simulink model "gm_comm8qamtxrxhdl"  (R2025b)
settings: Solver=FixedStepDiscrete  StartTime=0.0  StopTime=20000*qam_params.symbolPeriod  RelTol=1e-3
PreLoadFcn:
  | qam_params = comm8qamtxrxhdl_init;
InitFcn:
  | qam_params = comm8qamtxrxhdl_init;
libraries: simulink x16, hdlmdlgenlib x7, hdlsllib x7, commchan3 x1, commrflib2 x1, dspsigops x1, dsphdlsigops2 x1, dspmlti4 x1, commdigbbndam3 x1, commsequence2 x1
(part 2 of 3)

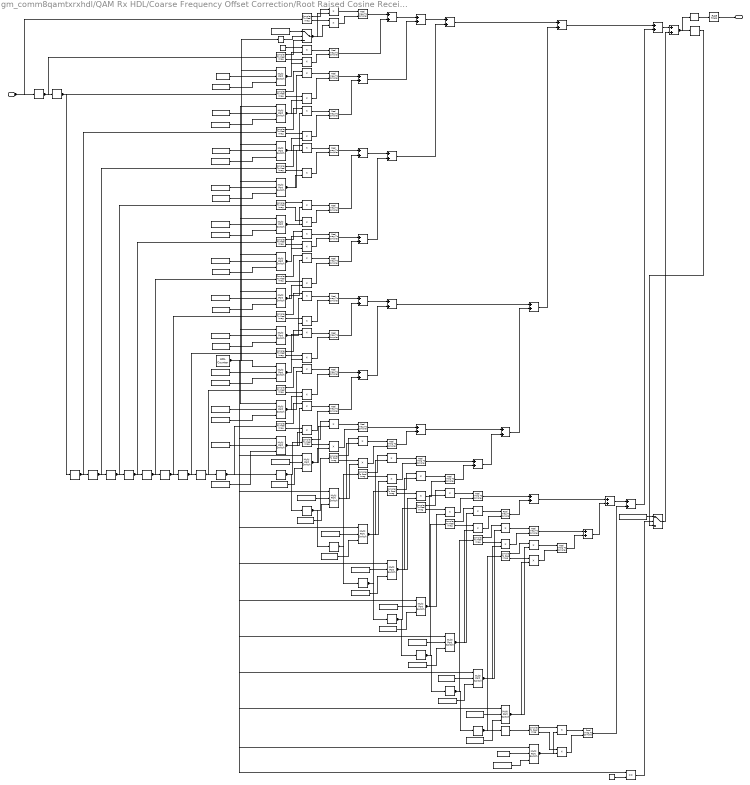
== system gm_comm8qamtxrxhdl/QAM Rx HDL/Coarse Frequency Offset Correction/Root Raised Cosine Receive Filter ==
  Root Raised Cosine Receive Filter_In : Inport  OutDataTypeStr=fixdt(1, 16, 15)  SampleTime=2.5e-07
      settings: SignalType=complex
  AddFeedback : Sum  OutDataTypeStr=fixdt(1, 16, 15)  SampleTime=2.5e-07
  Compare To Constant : simulink/Logic and Bit Operations/Compare To Constant  relop===  const=double(0)  OutDataTypeStr=boolean
  Constant : Constant  OutDataTypeStr=fixdt(0, 1, 0)  SampleTime=2.5e-07
  Constant1 : Constant  Value="fi(0,1,16,15,\"hex\",\"0000 + 0000 i\")"  OutDataTypeStr=fixdt(1, 16, 15)  SampleTime=2.5e-07
  Constant11 : Constant  Value=-0.0001678466796875  OutDataTypeStr=fixdt(1, 16, 16)  SampleTime=2.5e-07
  Constant12 : Constant  Value=0  OutDataTypeStr=fixdt(1, 16, 16)  SampleTime=2.5e-07
  Data Type Conversion : hdlmdlgenlib/Buffer
  Delay0 : Delay  DelayLength=double(1)  InitialCondition=0  SampleTime=2.5e-07
  Delay01 : Delay  DelayLength=double(2)  InitialCondition=0  SampleTime=2.5e-07
  Delay010 : Delay  DelayLength=double(2)  InitialCondition=0  SampleTime=2.5e-07
  Delay011 : Delay  DelayLength=double(2)  InitialCondition=0  SampleTime=2.5e-07
  Delay012 : Delay  DelayLength=double(2)  InitialCondition=0  SampleTime=2.5e-07
  Delay013 : Delay  DelayLength=double(2)  InitialCondition=0  SampleTime=2.5e-07
  Delay014 : Delay  DelayLength=double(2)  InitialCondition=0  SampleTime=2.5e-07
  Delay015 : Delay  DelayLength=double(2)  InitialCondition=0  SampleTime=2.5e-07
  Delay016 : Delay  DelayLength=double(2)  InitialCondition=0  SampleTime=2.5e-07
  Delay017 : Delay  DelayLength=double(2)  InitialCondition=0  SampleTime=2.5e-07
  Delay018 : Delay  DelayLength=double(2)  InitialCondition=0  SampleTime=2.5e-07
  Delay019 : Delay  DelayLength=double(2)  InitialCondition=0  SampleTime=2.5e-07
  Delay02 : Delay  DelayLength=double(2)  InitialCondition=0  SampleTime=2.5e-07
  Delay020 : Delay  DelayLength=double(1)  InitialCondition=0  SampleTime=2.5e-07
  Delay03 : Delay  DelayLength=double(2)  InitialCondition=0  SampleTime=2.5e-07
  Delay04 : Delay  DelayLength=double(2)  InitialCondition=0  SampleTime=2.5e-07
  Delay05 : Delay  DelayLength=double(2)  InitialCondition=0  SampleTime=2.5e-07
  Delay06 : Delay  DelayLength=double(2)  InitialCondition=0  SampleTime=2.5e-07
  Delay07 : Delay  DelayLength=double(2)  InitialCondition=0  SampleTime=2.5e-07
  Delay08 : Delay  DelayLength=double(2)  InitialCondition=0  SampleTime=2.5e-07
  Delay09 : Delay  DelayLength=double(2)  InitialCondition=0  SampleTime=2.5e-07
  HDL Counter : hdlsllib/Sources/HDL Counter  CountType=Count limited  CountInit=double(0)  CountStep=double(1)  CountMax=double(1)  CountFromType=Initial value  CountFrom=double(0)  CountResetPort=off  CountLoadPort=off  CountEnbPort=off  CountDirPort=off  CountHitOutputPort=off  CountDataType=Unsigned  CountWordLen=1  CountFracLen=0  CountSampTime=2.5e-07
  Multiport Switch{,1..19} (20 alike) : MultiPortSwitch  DataPortOrder=Zero-based contiguous  Inputs=2  DiagnosticForDefault=None  zeroidx=on  OutDataTypeStr=fixdt(1, 16, 16)  SampleTime=2.5e-07  SaturateOnIntegerOverflow=off  InputSameDT=off
  Product{10,101..109,1010..1041} (42 alike) : Product  Inputs=**  OutDataTypeStr=fixdt(1, 16, 15)  SampleTime=2.5e-07
  Product10_C2ReIm{,1..20} (21 alike) : ComplexToRealImag  SampleTime=2.5e-07
  Product10_ReIm2Complex{,1..20} (21 alike) : RealImagToComplex  SampleTime=2.5e-07
  Relational Operator : RelationalOperator  Operator===  OutDataTypeStr=fixdt(0, 1, 0)  SampleTime=2.5e-07  InputSameDT=off
  Switch : Switch  Criteria=u2 > Threshold  Threshold="fi(0,0,1,0,\"hex\",\"0\")"  OutDataTypeStr=fixdt(1, 16, 16)  SampleTime=2.5e-07  SaturateOnIntegerOverflow=off  InputSameDT=off
  Switch1 : Switch  Criteria=u2 > Threshold  Threshold="fi(0,0,1,0,\"hex\",\"0\")"  OutDataTypeStr=fixdt(1, 16, 15)  SampleTime=2.5e-07  SaturateOnIntegerOverflow=off  InputSameDT=off
  addtree{,1..19} (20 alike) : Sum  OutDataTypeStr=fixdt(1, 16, 15)  SampleTime=2.5e-07
  coeffSubVector : Constant  Value=-0.0041046142578125  OutDataTypeStr=fixdt(1, 16, 16)  SampleTime=2.5e-07
  coeffSubVector1 : Constant  Value=0.000762939453125  OutDataTypeStr=fixdt(1, 16, 16)  SampleTime=2.5e-07
  coeffSubVector10 : Constant  Value=-0.0391082763671875  OutDataTypeStr=fixdt(1, 16, 16)  SampleTime=2.5e-07
  coeffSubVector11 : Constant  Value=-0.026458740234375  OutDataTypeStr=fixdt(1, 16, 16)  SampleTime=2.5e-07
  coeffSubVector12 : Constant  Value=0.0391082763671875  OutDataTypeStr=fixdt(1, 16, 16)  SampleTime=2.5e-07
  coeffSubVector13 : Constant  Value=0.1443023681640625  OutDataTypeStr=fixdt(1, 16, 16)  SampleTime=2.5e-07
  coeffSubVector14 : Constant  Value=0.2430267333984375  OutDataTypeStr=fixdt(1, 16, 16)  SampleTime=2.5e-07
  coeffSubVector15 : Constant  Value=0.2834625244140625  OutDataTypeStr=fixdt(1, 16, 16)  SampleTime=2.5e-07
  coeffSubVector16 : Constant  Value=0.2430267333984375  OutDataTypeStr=fixdt(1, 16, 16)  SampleTime=2.5e-07
  coeffSubVector17 : Constant  Value=0.1443023681640625  OutDataTypeStr=fixdt(1, 16, 16)  SampleTime=2.5e-07
  coeffSubVector18 : Constant  Value=0.0391082763671875  OutDataTypeStr=fixdt(1, 16, 16)  SampleTime=2.5e-07
  coeffSubVector19 : Constant  Value=-0.026458740234375  OutDataTypeStr=fixdt(1, 16, 16)  SampleTime=2.5e-07
  coeffSubVector2 : Constant  Value=0.0041046142578125  OutDataTypeStr=fixdt(1, 16, 16)  SampleTime=2.5e-07
  coeffSubVector20 : Constant  Value=-0.0391082763671875  OutDataTypeStr=fixdt(1, 16, 16)  SampleTime=2.5e-07
  coeffSubVector21 : Constant  Value=-0.018707275390625  OutDataTypeStr=fixdt(1, 16, 16)  SampleTime=2.5e-07
  coeffSubVector{22,24,30,32} (4 alike) : Constant  Value=0.0038604736328125  OutDataTypeStr=fixdt(1, 16, 16)  SampleTime=2.5e-07
  coeffSubVector23 : Constant  Value=0.010589599609375  OutDataTypeStr=fixdt(1, 16, 16)  SampleTime=2.5e-07
  coeffSubVector25 : Constant  Value=-0.0037384033203125  OutDataTypeStr=fixdt(1, 16, 16)  SampleTime=2.5e-07
  coeffSubVector26 : Constant  Value=0.0041046142578125  OutDataTypeStr=fixdt(1, 16, 16)  SampleTime=2.5e-07
  coeffSubVector27 : Constant  Value=0.000762939453125  OutDataTypeStr=fixdt(1, 16, 16)  SampleTime=2.5e-07
  coeffSubVector28 : Constant  Value=-0.0041046142578125  OutDataTypeStr=fixdt(1, 16, 16)  SampleTime=2.5e-07
  coeffSubVector29 : Constant  Value=-0.0037384033203125  OutDataTypeStr=fixdt(1, 16, 16)  SampleTime=2.5e-07
  coeffSubVector3 : Constant  Value=0.0026702880859375  OutDataTypeStr=fixdt(1, 16, 16)  SampleTime=2.5e-07
  coeffSubVector31 : Constant  Value=0.010589599609375  OutDataTypeStr=fixdt(1, 16, 16)  SampleTime=2.5e-07
  coeffSubVector33 : Constant  Value=-0.018707275390625  OutDataTypeStr=fixdt(1, 16, 16)  SampleTime=2.5e-07
  coeffSubVector{4,6,34,36} (4 alike) : Constant  Value=-0.000946044921875  OutDataTypeStr=fixdt(1, 16, 16)  SampleTime=2.5e-07
  coeffSubVector35 : Constant  Value=-0.0025177001953125  OutDataTypeStr=fixdt(1, 16, 16)  SampleTime=2.5e-07
  coeffSubVector37 : Constant  Value=0.0026702880859375  OutDataTypeStr=fixdt(1, 16, 16)  SampleTime=2.5e-07
  coeffSubVector38 : Constant  Value=0.00146484375  OutDataTypeStr=fixdt(1, 16, 16)  SampleTime=2.5e-07
  coeffSubVector39 : Constant  Value=0.001251220703125  OutDataTypeStr=fixdt(1, 16, 16)  SampleTime=2.5e-07
  coeffSubVector5 : Constant  Value=-0.0025177001953125  OutDataTypeStr=fixdt(1, 16, 16)  SampleTime=2.5e-07
  coeffSubVector7 : Constant  Value=0.001251220703125  OutDataTypeStr=fixdt(1, 16, 16)  SampleTime=2.5e-07
  coeffSubVector8 : Constant  Value=0.00146484375  OutDataTypeStr=fixdt(1, 16, 16)  SampleTime=2.5e-07
  coeffSubVector9 : Constant  Value=-0.0001678466796875  OutDataTypeStr=fixdt(1, 16, 16)  SampleTime=2.5e-07
  rt : RateTransition  InitialCondition=double(0)  OutPortSampleTimeOpt=Multiple of input port sample time  OutPortSampleTimeMultiple=2
  Root Raised Cosine Receive Filter_out : Outport  OutDataTypeStr=fixdt(1, 16, 15)  SampleTime=5e-07
      settings: SignalType=complex
  wires:
  Switch1/1 -> AddFeedback/2
  Multiport Switch1/1 -> Product102/2, Product103/2
  Multiport Switch11/1 -> Product1022/2, Product1023/2
  Product1014/1 -> Product10_ReIm2Complex7/1
  Product1030/1 -> Product10_ReIm2Complex15/1
  coeffSubVector8/1 -> Multiport Switch4/2
  Product1040/1 -> Product10_ReIm2Complex20/1
  Constant1/1 -> Switch1/1
  Product1025/1 -> Product10_ReIm2Complex12/2
  Product1041/1 -> Product10_ReIm2Complex20/2
  Product1029/1 -> Product10_ReIm2Complex14/2
  Relational Operator/1 -> Switch1/2
  Product10_C2ReIm3/2 -> Product107/1
  Product10_C2ReIm19/1 -> Product1038/1
  Product10_C2ReIm3/1 -> Product106/1
  Product10_C2ReIm19/2 -> Product1039/1
  Product10_C2ReIm11/1 -> Product1022/1
  Product1037/1 -> Product10_ReIm2Complex18/2
  addtree3/1 -> addtree4/2
  Product105/1 -> Product10_ReIm2Complex2/2
  Product1021/1 -> Product10_ReIm2Complex10/2
  coeffSubVector5/1 -> Multiport Switch2/3
  Product10_ReIm2Complex12/1 -> addtree9/2
  Product10_C2ReIm18/1 -> Product1036/1
  Product10_C2ReIm2/2 -> Product105/1
  Product10_C2ReIm2/1 -> Product104/1
  Product10_C2ReIm18/2 -> Product1037/1
  Product10_C2ReIm12/1 -> Product1024/1
  Product10_C2ReIm4/1 -> Product108/1
  Product10_C2ReIm20/2 -> Product1041/1
  Product10_C2ReIm4/2 -> Product109/1
  Product10_C2ReIm20/1 -> Product1040/1
  Delay010/1 -> Delay011/1, Product10_C2ReIm8/1
  coeffSubVector39/1 -> Multiport Switch19/3
  Product1027/1 -> Product10_ReIm2Complex13/2
  Product1038/1 -> Product10_ReIm2Complex19/1
  Multiport Switch7/1 -> Product1015/2, Product1014/2
  coeffSubVector24/1 -> Multiport Switch12/2
  coeffSubVector16/1 -> Multiport Switch8/2
  Product1036/1 -> Product10_ReIm2Complex18/1
  Product1020/1 -> Product10_ReIm2Complex10/1
  coeffSubVector26/1 -> Multiport Switch13/2
  Multiport Switch/1 -> Product101/2, Product10/2
  Product10_ReIm2Complex17/1 -> addtree17/1
  coeffSubVector13/1 -> Multiport Switch6/3
  coeffSubVector21/1 -> Multiport Switch10/3
  Product1039/1 -> Product10_ReIm2Complex19/2
  Product10_ReIm2Complex7/1 -> addtree6/1
  HDL Counter/1 -> Multiport Switch/1, Relational Operator/1, Compare To Constant/1, Multiport Switch19/1, Multiport Switch17/1, Multiport Switch18/1, Multiport Switch14/1, Multiport Switch16/1, Multiport Switch5/1, Multiport Switch6/1, Multiport Switch8/1, Multiport Switch10/1, Multiport Switch13/1, Multiport Switch4/1, Multiport Switch2/1, Multiport Switch7/1, Multiport Switch3/1, Multiport Switch1/1, Multiport Switch12/1, Multiport Switch15/1, Multiport Switch11/1, Multiport Switch9/1
  Multiport Switch5/1 -> Product1011/2, Product1010/2
  addtree17/1 -> addtree18/2
  Product10_C2ReIm13/2 -> Product1027/1
  Product10_C2ReIm5/2 -> Product1011/1
  addtree4/1 -> AddFeedback/1
  Product1016/1 -> Product10_ReIm2Complex8/1
  Product1032/1 -> Product10_ReIm2Complex16/1
  Product103/1 -> Product10_ReIm2Complex1/2
  Product1035/1 -> Product10_ReIm2Complex17/2
  Product1019/1 -> Product10_ReIm2Complex9/2
  Product1028/1 -> Product10_ReIm2Complex14/1
  Product10_C2ReIm14/2 -> Product1029/1
  Delay012/1 -> Delay013/1, Product10_C2ReIm10/1
  Product1034/1 -> Product10_ReIm2Complex17/1
  Product10_C2ReIm15/1 -> Product1030/1
  addtree/1 -> addtree2/1
  Product10_C2ReIm15/2 -> Product1031/1
  Product10_C2ReIm7/2 -> Product1015/1
  coeffSubVector35/1 -> Multiport Switch17/3
  coeffSubVector28/1 -> Multiport Switch14/2
  Product10_C2ReIm9/1 -> Product1018/1
  Product10_C2ReIm1/2 -> Product103/1
  Product10_C2ReIm17/1 -> Product1034/1
  Product10_C2ReIm1/1 -> Product102/1
  Product10_C2ReIm17/2 -> Product1035/1
  Product1031/1 -> Product10_ReIm2Complex15/2
  Product1015/1 -> Product10_ReIm2Complex7/2
  coeffSubVector11/1 -> Multiport Switch5/3
  Product10_C2ReIm8/2 -> Product1017/1
  coeffSubVector19/1 -> Multiport Switch9/3
  Product10_C2ReIm/2 -> Product101/1
  Product10_C2ReIm16/1 -> Product1032/1
  Delay05/1 -> Product10_C2ReIm15/1, Delay06/1
  Product10_C2ReIm/1 -> Product10/1
  Product10_C2ReIm16/2 -> Product1033/1
  Product10_C2ReIm8/1 -> Product1016/1
  Product10_ReIm2Complex2/1 -> addtree1/1
  Root Raised Cosine Receive Filter_In/1 -> Delay0/1, Product10_C2ReIm20/1
  Product1033/1 -> Product10_ReIm2Complex16/2
  addtree18/1 -> addtree16/1
  Product1026/1 -> Product10_ReIm2Complex13/1
  addtree19/1 -> addtree18/1
  Product10_C2ReIm14/1 -> Product1028/1
  Product1017/1 -> Product10_ReIm2Complex8/2
  Product1023/1 -> Product10_ReIm2Complex11/2
  Product10_C2ReIm13/1 -> Product1026/1
  Multiport Switch17/1 -> Product1035/2, Product1034/2
  Product1024/1 -> Product10_ReIm2Complex12/1
  Product10_C2ReIm12/2 -> Product1025/1
  Product1022/1 -> Product10_ReIm2Complex11/1
  coeffSubVector29/1 -> Multiport Switch14/3
  Product10_C2ReIm11/2 -> Product1023/1
  coeffSubVector31/1 -> Multiport Switch15/3
  Product10_C2ReIm10/2 -> Product1021/1
  Product10_C2ReIm10/1 -> Product1020/1
  Delay09/1 -> Product10_C2ReIm7/1, Delay010/1
  Product1018/1 -> Product10_ReIm2Complex9/1
  Multiport Switch13/1 -> Product1027/2, Product1026/2
  Product10_C2ReIm9/2 -> Product1019/1
  Product10_C2ReIm7/1 -> Product1014/1
  Product1013/1 -> Product10_ReIm2Complex6/2
  Product1012/1 -> Product10_ReIm2Complex6/1
  addtree11/1 -> addtree12/2
  Product10_C2ReIm6/2 -> Product1013/1
  Product10_C2ReIm6/1 -> Product1012/1
  Product1011/1 -> Product10_ReIm2Complex5/2
  Product1010/1 -> Product10_ReIm2Complex5/1
  Product10_C2ReIm5/1 -> Product1010/1
  coeffSubVector27/1 -> Multiport Switch13/3
  Product109/1 -> Product10_ReIm2Complex4/2
  Product108/1 -> Product10_ReIm2Complex4/1
  Product107/1 -> Product10_ReIm2Complex3/2
  addtree7/1 -> addtree11/1
  Product106/1 -> Product10_ReIm2Complex3/1
  Product104/1 -> Product10_ReIm2Complex2/1
  addtree10/1 -> addtree11/2
  Product102/1 -> Product10_ReIm2Complex1/1
  coeffSubVector30/1 -> Multiport Switch15/2
  Product101/1 -> Product10_ReIm2Complex/2
  Product10/1 -> Product10_ReIm2Complex/1
  Product10_ReIm2Complex18/1 -> addtree17/2
  addtree16/1 -> addtree12/1
  coeffSubVector2/1 -> Multiport Switch1/2
  Product10_ReIm2Complex8/1 -> addtree6/2
  addtree14/1 -> addtree15/2
  Product10_ReIm2Complex16/1 -> addtree14/2
  Delay017/1 -> Delay018/1, Product10_C2ReIm2/1
  Product10_ReIm2Complex15/1 -> addtree14/1
  Product10_ReIm2Complex3/1 -> addtree1/2
  Multiport Switch3/1 -> Product106/2, Product107/2
  Product10_ReIm2Complex9/1 -> addtree8/1
  addtree13/1 -> addtree15/1
  Delay01/1 -> Product10_C2ReIm17/1, Delay02/1
  Product10_ReIm2Complex14/1 -> addtree13/2
  Product10_ReIm2Complex13/1 -> addtree13/1
  addtree6/1 -> addtree7/2
  addtree9/1 -> addtree10/2
  Product10_ReIm2Complex10/1 -> addtree8/2
  addtree5/1 -> addtree7/1
  Product10_ReIm2Complex6/1 -> addtree5/2
  Product10_ReIm2Complex5/1 -> addtree5/1
  addtree2/1 -> addtree3/1
  addtree1/1 -> addtree2/2
  Product10_ReIm2Complex1/1 -> addtree/2
  rt/1 -> Root Raised Cosine Receive Filter_out/1
  Compare To Constant/1 -> Switch/2
  Constant12/1 -> Switch/3
  Constant11/1 -> Switch/1
  Multiport Switch8/1 -> Product1017/2, Product1016/2
  Multiport Switch12/1 -> Product1025/2, Product1024/2
  Product10_ReIm2Complex20/1 -> addtree19/1
  coeffSubVector25/1 -> Multiport Switch12/3
  coeffSubVector38/1 -> Multiport Switch19/2
  coeffSubVector37/1 -> Multiport Switch18/3
  coeffSubVector36/1 -> Multiport Switch18/2
  Product10_ReIm2Complex11/1 -> addtree9/1
  coeffSubVector34/1 -> Multiport Switch17/2
  coeffSubVector3/1 -> Multiport Switch1/3
  coeffSubVector33/1 -> Multiport Switch16/3
  coeffSubVector32/1 -> Multiport Switch16/2
  coeffSubVector14/1 -> Multiport Switch7/2
  coeffSubVector23/1 -> Multiport Switch11/3
  Multiport Switch9/1 -> Product1019/2, Product1018/2
  coeffSubVector22/1 -> Multiport Switch11/2
  coeffSubVector12/1 -> Multiport Switch6/2
  coeffSubVector20/1 -> Multiport Switch10/2
  coeffSubVector18/1 -> Multiport Switch9/2
  Delay03/1 -> Delay04/1, Product10_C2ReIm13/1
  coeffSubVector17/1 -> Multiport Switch8/3
  coeffSubVector15/1 -> Multiport Switch7/3
  Multiport Switch10/1 -> Product1021/2, Product1020/2
  Data Type Conversion/1 -> rt/1
  coeffSubVector10/1 -> Multiport Switch5/2
  coeffSubVector9/1 -> Multiport Switch4/3
  coeffSubVector7/1 -> Multiport Switch3/3
  coeffSubVector6/1 -> Multiport Switch3/2
  Multiport Switch6/1 -> Product1012/2, Product1013/2
  AddFeedback/1 -> Data Type Conversion/1, Delay020/1
  coeffSubVector4/1 -> Multiport Switch2/2
  coeffSubVector1/1 -> Multiport Switch/3
  coeffSubVector/1 -> Multiport Switch/2
  Constant/1 -> Relational Operator/2
  Delay019/1 -> Product10_C2ReIm4/1
  Switch/1 -> Product1041/2, Product1040/2
  Multiport Switch19/1 -> Product1039/2, Product1038/2
  Multiport Switch18/1 -> Product1037/2, Product1036/2
  Multiport Switch16/1 -> Product1033/2, Product1032/2
  Multiport Switch15/1 -> Product1031/2, Product1030/2
  Multiport Switch14/1 -> Product1029/2, Product1028/2
  Delay011/1 -> Delay012/1, Product10_C2ReIm9/1
  Delay013/1 -> Delay014/1, Product10_C2ReIm11/1
  Multiport Switch4/1 -> Product109/2, Product108/2
  Delay015/1 -> Delay016/1, Product10_C2ReIm/1
  Multiport Switch2/1 -> Product105/2, Product104/2
  Delay018/1 -> Product10_C2ReIm3/1, Delay019/1
  Delay016/1 -> Product10_C2ReIm1/1, Delay017/1
  Delay014/1 -> Product10_C2ReIm12/1, Delay015/1
  Delay06/1 -> Product10_C2ReIm16/1, Delay07/1
  Delay08/1 -> Product10_C2ReIm6/1, Delay09/1
  Delay07/1 -> Product10_C2ReIm5/1, Delay08/1
  Delay04/1 -> Product10_C2ReIm14/1, Delay05/1
  Delay02/1 -> Product10_C2ReIm18/1, Delay03/1
  Delay0/1 -> Product10_C2ReIm19/1, Delay01/1
  addtree15/1 -> addtree16/2
  addtree12/1 -> addtree4/1
  Product10_ReIm2Complex19/1 -> addtree19/2
  addtree8/1 -> addtree10/1
  Product10_ReIm2Complex/1 -> addtree/1
  Product10_ReIm2Complex4/1 -> addtree3/2
  Delay020/1 -> Switch1/3

== system gm_comm8qamtxrxhdl/QAM Rx HDL/Demodulate/Rectangular QAM Demodulator Baseband ==
  u : Inport  OutDataTypeStr=fixdt(1, 16, 12)  PortDimensions=1  SampleTime=5e-07
      settings: SignalType=complex
  Rectangular QAM Demodulator Baseband : MATLAB Function  TreatAsAtomicUnit=on
  y : Outport  SampleTime=5e-07
  wires:
  u/1 -> Rectangular QAM Demodulator Baseband/1(u)
  Rectangular QAM Demodulator Baseband/1(y) -> y/1

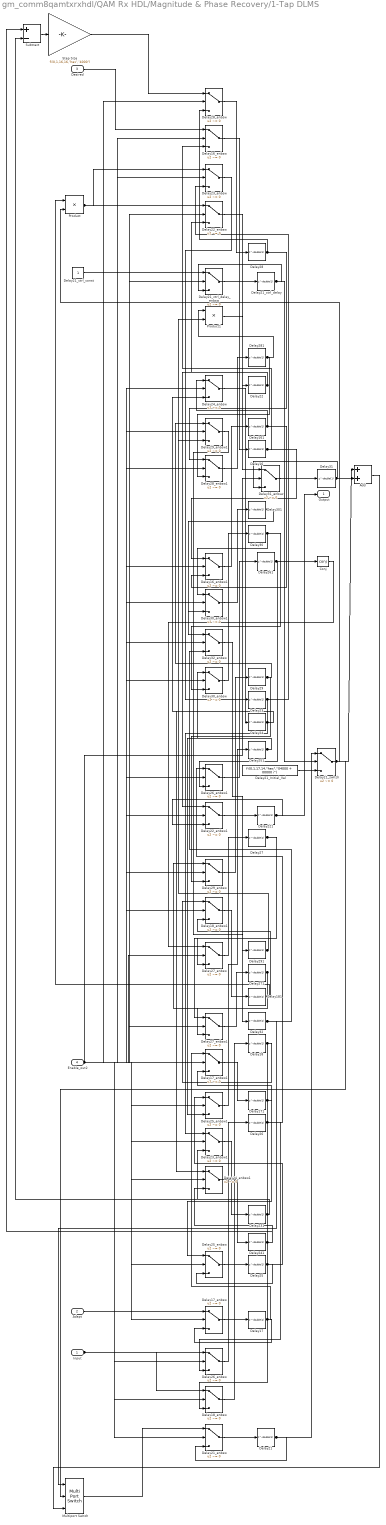
== system gm_comm8qamtxrxhdl/QAM Rx HDL/Magnitude & Phase Recovery/1-Tap DLMS ==
  Input : Inport  OutDataTypeStr=fixdt(1, 16, 15)  PortDimensions=1  SampleTime=5e-07
      settings: SignalType=complex
  Adapt : Inport  Port=2  OutDataTypeStr=boolean  PortDimensions=1  SampleTime=5e-07
  Desired : Inport  Port=3  OutDataTypeStr=fixdt(1, 16, 15)  PortDimensions=1  SampleTime=5e-07
      settings: SignalType=complex
  Enable_out2 : Inport  Port=4  OutDataTypeStr=boolean  SampleTime=5e-07
  Add : Sum  OutDataTypeStr=fixdt(1, 17, 14)  AccumDataTypeStr=fixdt(1, 19, 15)  SampleTime=5e-07
  Conj : Math  Operator=conj  SignedPower=on  OutDataTypeStr=fixdt(1, 16, 15)
  Delay{16..18,21..32,161,171,181,221,231,241,251,261,271,281,291,301} (27 alike) : Delay  DelayLength=double(1)  InitialCondition=0
  Delay16_enbsw : Switch  Criteria=u2 ~= 0  Threshold=double(0)  OutDataTypeStr=fixdt(1, 16, 15)  SampleTime=5e-07  SaturateOnIntegerOverflow=off  InputSameDT=off
  Delay16_enbsw1 : Switch  Criteria=u2 ~= 0  Threshold=double(0)  OutDataTypeStr=fixdt(1, 16, 15)  SampleTime=5e-07  SaturateOnIntegerOverflow=off  InputSameDT=off
  Delay17_enbsw : Switch  Criteria=u2 ~= 0  Threshold=double(0)  OutDataTypeStr=boolean  SampleTime=5e-07  SaturateOnIntegerOverflow=off  InputSameDT=off
  Delay17_enbsw1 : Switch  Criteria=u2 ~= 0  Threshold=double(0)  OutDataTypeStr=boolean  SampleTime=5e-07  SaturateOnIntegerOverflow=off  InputSameDT=off
  Delay18_enbsw : Switch  Criteria=u2 ~= 0  Threshold=double(0)  OutDataTypeStr=fixdt(1, 16, 15)  SampleTime=5e-07  SaturateOnIntegerOverflow=off  InputSameDT=off
  Delay18_enbsw1 : Switch  Criteria=u2 ~= 0  Threshold=double(0)  OutDataTypeStr=fixdt(1, 16, 15)  SampleTime=5e-07  SaturateOnIntegerOverflow=off  InputSameDT=off
  Delay21_Initial_Val : Constant  Value="fi(0,1,17,14,\"hex\",\"04000 + 00000 i\")"  OutDataTypeStr=fixdt(1, 17, 14)  SampleTime=5e-07
  Delay21_ctrl_const : Constant  OutDataTypeStr=boolean  SampleTime=5e-07
  Delay21_ctrl_delay : Delay  DelayLength=double(1)  InitialCondition=0
  Delay21_ctrl_delay_enbsw : Switch  Criteria=u2 ~= 0  Threshold=double(0)  OutDataTypeStr=boolean  SampleTime=5e-07  SaturateOnIntegerOverflow=off  InputSameDT=off
  Delay21_enbsw : Switch  Criteria=u2 ~= 0  Threshold=double(0)  OutDataTypeStr=fixdt(1, 17, 14)  SampleTime=5e-07  SaturateOnIntegerOverflow=off  InputSameDT=off
  Delay21_switch : Switch  Criteria=u2 ~= 0  Threshold=double(0)  OutDataTypeStr=fixdt(1, 17, 14)  SampleTime=5e-07  SaturateOnIntegerOverflow=off  InputSameDT=off
  Delay22_enbsw : Switch  Criteria=u2 ~= 0  Threshold=double(0)  OutDataTypeStr=fixdt(1, 16, 14)  SampleTime=5e-07  SaturateOnIntegerOverflow=off  InputSameDT=off
  Delay22_enbsw1 : Switch  Criteria=u2 ~= 0  Threshold=double(0)  OutDataTypeStr=fixdt(1, 16, 14)  SampleTime=5e-07  SaturateOnIntegerOverflow=off  InputSameDT=off
  Delay23_enbsw : Switch  Criteria=u2 ~= 0  Threshold=double(0)  OutDataTypeStr=fixdt(1, 16, 14)  SampleTime=5e-07  SaturateOnIntegerOverflow=off  InputSameDT=off
  Delay23_enbsw1 : Switch  Criteria=u2 ~= 0  Threshold=double(0)  OutDataTypeStr=fixdt(1, 16, 14)  SampleTime=5e-07  SaturateOnIntegerOverflow=off  InputSameDT=off
  Delay24_enbsw : Switch  Criteria=u2 ~= 0  Threshold=double(0)  OutDataTypeStr=fixdt(1, 16, 15)  SampleTime=5e-07  SaturateOnIntegerOverflow=off  InputSameDT=off
  Delay24_enbsw1 : Switch  Criteria=u2 ~= 0  Threshold=double(0)  OutDataTypeStr=fixdt(1, 16, 15)  SampleTime=5e-07  SaturateOnIntegerOverflow=off  InputSameDT=off
  Delay25_enbsw : Switch  Criteria=u2 ~= 0  Threshold=double(0)  OutDataTypeStr=boolean  SampleTime=5e-07  SaturateOnIntegerOverflow=off  InputSameDT=off
  Delay25_enbsw1 : Switch  Criteria=u2 ~= 0  Threshold=double(0)  OutDataTypeStr=boolean  SampleTime=5e-07  SaturateOnIntegerOverflow=off  InputSameDT=off
  Delay26_enbsw : Switch  Criteria=u2 ~= 0  Threshold=double(0)  OutDataTypeStr=fixdt(1, 16, 15)  SampleTime=5e-07  SaturateOnIntegerOverflow=off  InputSameDT=off
  Delay26_enbsw1 : Switch  Criteria=u2 ~= 0  Threshold=double(0)  OutDataTypeStr=fixdt(1, 16, 15)  SampleTime=5e-07  SaturateOnIntegerOverflow=off  InputSameDT=off
  Delay27_enbsw : Switch  Criteria=u2 ~= 0  Threshold=double(0)  OutDataTypeStr=fixdt(1, 16, 15)  SampleTime=5e-07  SaturateOnIntegerOverflow=off  InputSameDT=off
  Delay27_enbsw1 : Switch  Criteria=u2 ~= 0  Threshold=double(0)  OutDataTypeStr=fixdt(1, 16, 15)  SampleTime=5e-07  SaturateOnIntegerOverflow=off  InputSameDT=off
  Delay28_enbsw : Switch  Criteria=u2 ~= 0  Threshold=double(0)  OutDataTypeStr=fixdt(1, 16, 15)  SampleTime=5e-07  SaturateOnIntegerOverflow=off  InputSameDT=off
  Delay28_enbsw1 : Switch  Criteria=u2 ~= 0  Threshold=double(0)  OutDataTypeStr=fixdt(1, 16, 15)  SampleTime=5e-07  SaturateOnIntegerOverflow=off  InputSameDT=off
  Delay29_enbsw : Switch  Criteria=u2 ~= 0  Threshold=double(0)  OutDataTypeStr=fixdt(1, 16, 15)  SampleTime=5e-07  SaturateOnIntegerOverflow=off  InputSameDT=off
  Delay29_enbsw1 : Switch  Criteria=u2 ~= 0  Threshold=double(0)  OutDataTypeStr=fixdt(1, 16, 15)  SampleTime=5e-07  SaturateOnIntegerOverflow=off  InputSameDT=off
  Delay30_enbsw : Switch  Criteria=u2 ~= 0  Threshold=double(0)  OutDataTypeStr=boolean  SampleTime=5e-07  SaturateOnIntegerOverflow=off  InputSameDT=off
  Delay30_enbsw1 : Switch  Criteria=u2 ~= 0  Threshold=double(0)  OutDataTypeStr=boolean  SampleTime=5e-07  SaturateOnIntegerOverflow=off  InputSameDT=off
  Delay31_enbsw : Switch  Criteria=u2 ~= 0  Threshold=double(0)  OutDataTypeStr=fixdt(1, 16, 15)  SampleTime=5e-07  SaturateOnIntegerOverflow=off  InputSameDT=off
  Delay32_enbsw : Switch  Criteria=u2 ~= 0  Threshold=double(0)  OutDataTypeStr=boolean  SampleTime=5e-07  SaturateOnIntegerOverflow=off  InputSameDT=off
  Multiport Switch : MultiPortSwitch  DataPortOrder=Zero-based contiguous  Inputs=2  DiagnosticForDefault=None  zeroidx=on  OutDataTypeStr=fixdt(1, 17, 14)  SampleTime=5e-07  SaturateOnIntegerOverflow=off  InputSameDT=off
  Product : Product  Inputs=**  OutDataTypeStr=fixdt(1, 16, 14)  SampleTime=5e-07
  Product1 : Product  Inputs=**  OutDataTypeStr=fixdt(1, 16, 15)  SampleTime=5e-07
  Step Size : Gain  Gain="fi(0,1,16,16,\"hex\",\"4000\")"  ParamDataTypeStr=fixdt(1, 16, 16)  OutDataTypeStr=fixdt(1, 16, 15)  SampleTime=5e-07
  Subtract : Sum  Inputs=+-  OutDataTypeStr=fixdt(1, 16, 14)  AccumDataTypeStr=fixdt(1, 16, 14)  SampleTime=5e-07
  Output : Outport  SampleTime=5e-07  VectorParamsAs1DForOutWhenUnconnected=off
  wires:
  Input/1 -> Delay18_enbsw/1, Delay26_enbsw/1
  Subtract/1 -> Step Size/1
  Delay22_enbsw/1 -> Delay22/1
  Desired/1 -> Delay16_enbsw/1
  Adapt/1 -> Delay17_enbsw/1
  Step Size/1 -> Delay28_enbsw/1
  Product/1 -> Delay23_enbsw/1, Delay22_enbsw/1
  Delay221/1 -> Delay22_enbsw1/3, Output/1
  Delay21_Initial_Val/1 -> Delay21_switch/3
  Delay21_ctrl_const/1 -> Delay21_ctrl_delay_enbsw/1
  Delay22/1 -> Delay22_enbsw/3, Delay22_enbsw1/1
  Enable_out2/1 -> Delay31_enbsw/2, Delay22_enbsw1/2, Delay32_enbsw/2, Delay26_enbsw/2, Delay26_enbsw1/2, Delay29_enbsw/2, Delay27_enbsw1/2, Delay24_enbsw1/2, Delay27_enbsw/2, Delay16_enbsw/2, Delay23_enbsw/2, Delay21_enbsw/2, Delay30_enbsw/2, Delay16_enbsw1/2, Delay22_enbsw/2, Delay17_enbsw1/2, Delay25_enbsw/2, Delay17_enbsw/2, Delay23_enbsw1/2, Delay18_enbsw/2, Delay21_ctrl_delay_enbsw/2, Delay28_enbsw/2, Delay30_enbsw1/2, Delay29_enbsw1/2, Delay18_enbsw1/2, Delay28_enbsw1/2, Delay24_enbsw/2, Delay25_enbsw1/2
  Multiport Switch/1 -> Delay21_enbsw/1
  Delay28_enbsw/1 -> Delay28/1
  Delay16_enbsw/1 -> Delay16/1
  Delay23_enbsw/1 -> Delay23/1
  Delay21_ctrl_delay_enbsw/1 -> Delay21_ctrl_delay/1
  Product1/1 -> Delay31_enbsw/1
  Delay24_enbsw/1 -> Delay24/1
  Delay29_enbsw1/1 -> Delay291/1
  Delay28_enbsw1/1 -> Delay281/1
  Delay16_enbsw1/1 -> Delay161/1
  Delay30_enbsw1/1 -> Delay301/1
  Delay32_enbsw/1 -> Delay32/1
  Delay30_enbsw/1 -> Delay30/1
  Delay26_enbsw1/1 -> Delay261/1
  Delay22_enbsw1/1 -> Delay221/1
  Delay29_enbsw/1 -> Delay29/1
  Delay18_enbsw1/1 -> Delay181/1
  Delay27_enbsw/1 -> Delay27/1
  Delay27_enbsw1/1 -> Delay271/1
  Delay17_enbsw1/1 -> Delay171/1
  Delay25_enbsw1/1 -> Delay251/1
  Delay231/1 -> Subtract/2, Delay23_enbsw1/3
  Delay23_enbsw1/1 -> Delay231/1
  Delay24_enbsw1/1 -> Delay241/1
  Delay25_enbsw/1 -> Delay25/1
  Delay17_enbsw/1 -> Delay17/1
  Delay26_enbsw/1 -> Delay26/1
  Delay18_enbsw/1 -> Delay18/1
  Delay21_enbsw/1 -> Delay21/1
  Delay28/1 -> Delay28_enbsw/3, Delay28_enbsw1/1
  Delay21_ctrl_delay/1 -> Delay21_ctrl_delay_enbsw/3, Delay21_switch/2
  Delay281/1 -> Product1/1, Delay28_enbsw1/3
  Delay161/1 -> Delay24_enbsw/1, Delay16_enbsw1/3
  Delay16/1 -> Delay16_enbsw/3, Delay16_enbsw1/1
  Delay31_enbsw/1 -> Delay31/1
  Delay301/1 -> Delay32_enbsw/1, Delay30_enbsw1/3
  Delay30/1 -> Delay30_enbsw1/1, Delay30_enbsw/3
  Delay261/1 -> Delay26_enbsw1/3, Conj/1
  Delay29/1 -> Delay29_enbsw/3, Delay29_enbsw1/1
  Delay23/1 -> Delay23_enbsw/3, Delay23_enbsw1/1
  Delay24/1 -> Delay24_enbsw1/1, Delay24_enbsw/3
  Delay251/1 -> Delay25_enbsw1/3, Delay30_enbsw/1
  Delay27/1 -> Delay27_enbsw1/1, Delay27_enbsw/3
  Delay291/1 -> Delay29_enbsw1/3, Product1/2
  Delay271/1 -> Delay27_enbsw1/3, Delay29_enbsw/1
  Delay181/1 -> Delay18_enbsw1/3, Product/1
  Delay32/1 -> Multiport Switch/1, Delay32_enbsw/3
  Delay18/1 -> Delay18_enbsw1/1, Delay18_enbsw/3
  Delay171/1 -> Delay17_enbsw1/3, Delay25_enbsw/1
  Delay26/1 -> Delay26_enbsw1/1, Delay26_enbsw/3
  Delay241/1 -> Subtract/1, Delay24_enbsw1/3
  Delay25/1 -> Delay25_enbsw1/1, Delay25_enbsw/3
  Delay17/1 -> Delay17_enbsw/3, Delay17_enbsw1/1
  Delay21/1 -> Delay21_enbsw/3, Delay21_switch/1
  Delay31/1 -> Delay31_enbsw/3, Add/2
  Conj/1 -> Delay27_enbsw/1
  Delay21_switch/1 -> Multiport Switch/2, Product/2, Add/1
  Add/1 -> Multiport Switch/3

== system gm_comm8qamtxrxhdl/QAM Rx HDL/Magnitude & Phase Recovery/Desired Signal Source ==
  Enable : Inport  OutDataTypeStr=boolean  PortDimensions=1  SampleTime=5e-07
  Enable_out2 : Inport  Port=2  OutDataTypeStr=boolean  SampleTime=5e-07
  HDL Counter2 : Delay  DelayLength=double(1)  InitialCondition=0
  HDL Counter2_enbsw : Switch  Criteria=u2 ~= 0  Threshold=double(0)  OutDataTypeStr=uint8  SampleTime=5e-07  SaturateOnIntegerOverflow=off  InputSameDT=off
  adder : Sum  OutDataTypeStr=uint8  AccumDataTypeStr=uint8  SampleTime=5e-07
  compare : simulink/Logic and Bit Operations/Compare To Constant  relop===  const="fi(0,0,8,0,\"hex\",\"0d\")"  OutDataTypeStr=boolean
  countFrom : Constant  Value=0  VectorParams1D=off  OutDataTypeStr=uint8  SampleTime=5e-07
  data lookup : LookupNDDirect  NumberOfTableDimensions=1  Table="reshape(complex(double([0.75+0.25i;0.75+0.25i;0.75+0.25i;0.75+0.25i;0.75+0.25i;-0.75-0.25i;-0.75-0.25i;0.75+0.25i;0.75+0.25i;-0.75-0.25i;0.75+0.25i;-0.75-0.25i;0.75+0.25i;0.75+0.25i])), [1  14])"  DiagnosticForOutOfRangeInput=Error  SampleTime=5e-07  TableDataTypeStr=fixdt(1,16,15)
  step_value : Constant  VectorParams1D=off  OutDataTypeStr=uint8  SampleTime=5e-07
  switch : Switch  Criteria=u2 ~= 0  Threshold="fi(0,0,1,0,\"hex\",\"0\")"  OutDataTypeStr=uint8  SampleTime=5e-07  SaturateOnIntegerOverflow=off  InputSameDT=off
  switchEnable : MultiPortSwitch  DataPortOrder=Zero-based contiguous  Inputs=2  DiagnosticForDefault=None  zeroidx=on  OutDataTypeStr=uint8  SampleTime=5e-07  SaturateOnIntegerOverflow=off  InputSameDT=off
  Output : Outport  SampleTime=5e-07  VectorParamsAs1DForOutWhenUnconnected=off
  wires:
  Enable/1 -> switchEnable/1
  switchEnable/1 -> HDL Counter2_enbsw/1
  compare/1 -> switch/2
  HDL Counter2/1 -> HDL Counter2_enbsw/3, switchEnable/2, compare/1, adder/1, data lookup/1
  Enable_out2/1 -> HDL Counter2_enbsw/2
  switch/1 -> switchEnable/3
  HDL Counter2_enbsw/1 -> HDL Counter2/1
  data lookup/1 -> Output/1
  step_value/1 -> adder/2
  countFrom/1 -> switch/1
  adder/1 -> switch/3

== system gm_comm8qamtxrxhdl/QAM Rx HDL/Magnitude & Phase Recovery/MATLAB Function3 ==
  in0 : Inport  OutDataTypeStr=boolean  SampleTime=5e-07
  Enable_out2 : EnablePort  OutDataTypeStr=boolean
  MATLAB Function3 : Subsystem
  out0 : Outport  OutDataTypeStr=boolean  SampleTime=5e-07  InitialOutput=0
  out1 : Outport  Port=2  OutDataTypeStr=boolean  SampleTime=5e-07  InitialOutput=0
  wires:
  MATLAB Function3/1(dvalid) -> out0/1
  in0/1 -> MATLAB Function3/1(enable)
  MATLAB Function3/2(isPreamble) -> out1/1

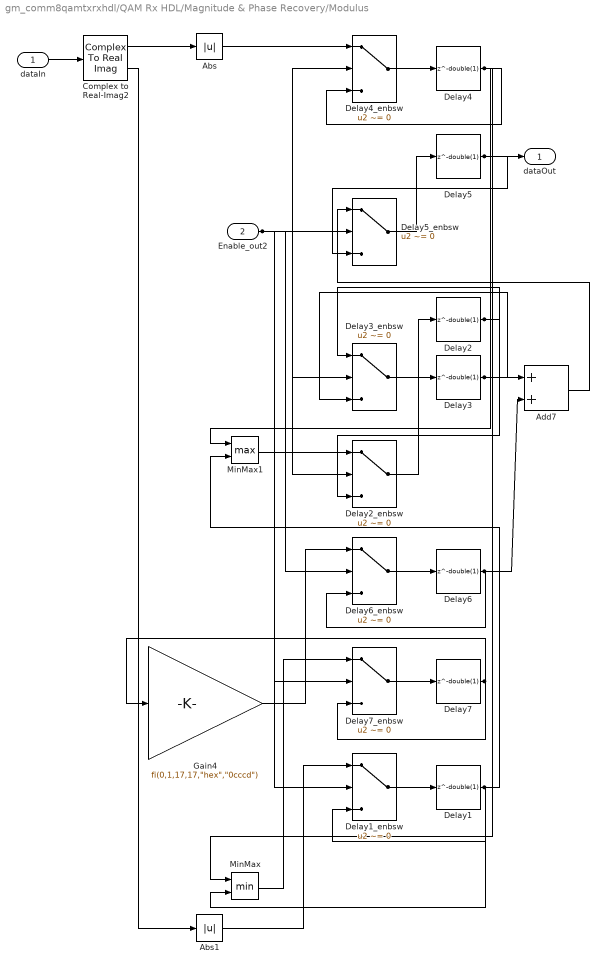
== system gm_comm8qamtxrxhdl/QAM Rx HDL/Magnitude & Phase Recovery/Modulus ==
  dataIn : Inport  OutDataTypeStr=fixdt(1, 17, 15)  PortDimensions=1  SampleTime=5e-07
      settings: SignalType=complex
  Enable_out2 : Inport  Port=2  OutDataTypeStr=boolean  SampleTime=5e-07
  Abs : Abs  SampleTime=5e-07  OutDataTypeStr=fixdt(1, 17, 15)  SaturateOnIntegerOverflow=off
  Abs1 : Abs  SampleTime=5e-07  OutDataTypeStr=fixdt(1, 17, 15)  SaturateOnIntegerOverflow=off
  Add7 : Sum  OutDataTypeStr=fixdt(1, 18, 15)  AccumDataTypeStr=fixdt(1, 18, 15)  SampleTime=5e-07
  Complex to Real-Imag2 : ComplexToRealImag  SampleTime=5e-07
  Delay{1..7} (7 alike) : Delay  DelayLength=double(1)  InitialCondition=0
  Delay1_enbsw : Switch  Criteria=u2 ~= 0  Threshold=double(0)  OutDataTypeStr=fixdt(1, 17, 15)  SampleTime=5e-07  SaturateOnIntegerOverflow=off  InputSameDT=off
  Delay2_enbsw : Switch  Criteria=u2 ~= 0  Threshold=double(0)  OutDataTypeStr=fixdt(1, 17, 15)  SampleTime=5e-07  SaturateOnIntegerOverflow=off  InputSameDT=off
  Delay3_enbsw : Switch  Criteria=u2 ~= 0  Threshold=double(0)  OutDataTypeStr=fixdt(1, 17, 15)  SampleTime=5e-07  SaturateOnIntegerOverflow=off  InputSameDT=off
  Delay4_enbsw : Switch  Criteria=u2 ~= 0  Threshold=double(0)  OutDataTypeStr=fixdt(1, 17, 15)  SampleTime=5e-07  SaturateOnIntegerOverflow=off  InputSameDT=off
  Delay5_enbsw : Switch  Criteria=u2 ~= 0  Threshold=double(0)  OutDataTypeStr=fixdt(1, 18, 15)  SampleTime=5e-07  SaturateOnIntegerOverflow=off  InputSameDT=off
  Delay6_enbsw : Switch  Criteria=u2 ~= 0  Threshold=double(0)  OutDataTypeStr=fixdt(1, 16, 15)  SampleTime=5e-07  SaturateOnIntegerOverflow=off  InputSameDT=off
  Delay7_enbsw : Switch  Criteria=u2 ~= 0  Threshold=double(0)  OutDataTypeStr=fixdt(1, 17, 15)  SampleTime=5e-07  SaturateOnIntegerOverflow=off  InputSameDT=off
  Gain4 : Gain  Gain="fi(0,1,17,17,\"hex\",\"0cccd\")"  ParamDataTypeStr=fixdt(1, 17, 17)  OutDataTypeStr=fixdt(1, 16, 15)  SampleTime=5e-07
  MinMax : MinMax  Inputs=2  OutDataTypeStr=fixdt(1, 17, 15)
  MinMax1 : MinMax  Function=max  Inputs=2  OutDataTypeStr=fixdt(1, 17, 15)
  dataOut : Outport  SampleTime=5e-07  VectorParamsAs1DForOutWhenUnconnected=off
  wires:
  dataIn/1 -> Complex to Real-Imag2/1
  Add7/1 -> Delay5_enbsw/1
  Complex to Real-Imag2/1 -> Abs/1
  Delay4_enbsw/1 -> Delay4/1
  MinMax/1 -> Delay7_enbsw/1
  Complex to Real-Imag2/2 -> Abs1/1
  Gain4/1 -> Delay6_enbsw/1
  Delay4/1 -> MinMax1/1, Delay4_enbsw/3, MinMax/1
  Abs/1 -> Delay4_enbsw/1
  Enable_out2/1 -> Delay4_enbsw/2, Delay3_enbsw/2, Delay1_enbsw/2, Delay7_enbsw/2, Delay6_enbsw/2, Delay2_enbsw/2, Delay5_enbsw/2
  MinMax1/1 -> Delay2_enbsw/1
  Abs1/1 -> Delay1_enbsw/1
  Delay5_enbsw/1 -> Delay5/1
  Delay3_enbsw/1 -> Delay3/1
  Delay2_enbsw/1 -> Delay2/1
  Delay6_enbsw/1 -> Delay6/1
  Delay7_enbsw/1 -> Delay7/1
  Delay1_enbsw/1 -> Delay1/1
  Delay5/1 -> Delay5_enbsw/3, dataOut/1
  Delay2/1 -> Delay3_enbsw/1, Delay2_enbsw/3
  Delay3/1 -> Delay3_enbsw/3, Add7/1
  Delay6/1 -> Delay6_enbsw/3, Add7/2
  Delay7/1 -> Gain4/1, Delay7_enbsw/3
  Delay1/1 -> Delay1_enbsw/3, MinMax1/2, MinMax/2

== system gm_comm8qamtxrxhdl/QAM Rx HDL/Magnitude & Phase Recovery/Preamble Matched Filter ==
  dataIn : Inport  OutDataTypeStr=fixdt(1, 16, 15)  PortDimensions=1  SampleTime=5e-07
      settings: SignalType=complex
  Enable_out2 : Inport  Port=2  OutDataTypeStr=boolean  SampleTime=5e-07
  Add2 : Sum  OutDataTypeStr=fixdt(1, 17, 15)  AccumDataTypeStr=fixdt(1, 17, 15)  SampleTime=5e-07
  Add3 : Sum  Inputs=+-  OutDataTypeStr=fixdt(1, 17, 15)  AccumDataTypeStr=fixdt(1, 17, 15)  SampleTime=5e-07
  Complex to Real-Imag2 : ComplexToRealImag  SampleTime=5e-07
  Delay{1..4} (4 alike) : Delay  DelayLength=double(1)  InitialCondition=0
  Delay1_enbsw : Switch  Criteria=u2 ~= 0  Threshold=double(0)  OutDataTypeStr=fixdt(1, 17, 15)  SampleTime=5e-07  SaturateOnIntegerOverflow=off  InputSameDT=off
  Delay2_enbsw : Switch  Criteria=u2 ~= 0  Threshold=double(0)  OutDataTypeStr=fixdt(1, 17, 15)  SampleTime=5e-07  SaturateOnIntegerOverflow=off  InputSameDT=off
  Delay3_enbsw : Switch  Criteria=u2 ~= 0  Threshold=double(0)  OutDataTypeStr=fixdt(1, 17, 15)  SampleTime=5e-07  SaturateOnIntegerOverflow=off  InputSameDT=off
  Delay4_enbsw : Switch  Criteria=u2 ~= 0  Threshold=double(0)  OutDataTypeStr=fixdt(1, 17, 15)  SampleTime=5e-07  SaturateOnIntegerOverflow=off  InputSameDT=off
  Discrete FIR Filter3 : Subsystem
  Discrete FIR Filter4 : Subsystem
  Real-Imag to Complex2 : RealImagToComplex  ConstantPart="fi(0,1,17,15,\"hex\",\"00000\")"  SampleTime=5e-07
  dataOut : Outport  SampleTime=5e-07  VectorParamsAs1DForOutWhenUnconnected=off
  wires:
  Add2/1 -> Delay4_enbsw/1
  Complex to Real-Imag2/1 -> Add2/1, Add3/1
  dataIn/1 -> Complex to Real-Imag2/1
  Complex to Real-Imag2/2 -> Add3/2, Add2/2
  Add3/1 -> Delay1_enbsw/1
  Delay1_enbsw/1 -> Delay1/1
  Enable_out2/1 -> Delay2_enbsw/2, Delay3_enbsw/2, Discrete FIR Filter3/2(Enable_out2), Delay4_enbsw/2, Discrete FIR Filter4/2(Enable_out2), Delay1_enbsw/2
  Discrete FIR Filter4/1(Discrete FIR Filter4_out) -> Delay3_enbsw/1
  Delay3_enbsw/1 -> Delay3/1
  Discrete FIR Filter3/1(Discrete FIR Filter3_out) -> Delay2_enbsw/1
  Delay4_enbsw/1 -> Delay4/1
  Delay1/1 -> Discrete FIR Filter4/1(Discrete FIR Filter4_in), Delay1_enbsw/3
  Delay2_enbsw/1 -> Delay2/1
  Delay4/1 -> Discrete FIR Filter3/1(Discrete FIR Filter3_in), Delay4_enbsw/3
  Delay2/1 -> Real-Imag to Complex2/1, Delay2_enbsw/3
  Delay3/1 -> Delay3_enbsw/3, Real-Imag to Complex2/2
  Real-Imag to Complex2/1 -> dataOut/1

== system gm_comm8qamtxrxhdl/QAM Rx HDL/Timing Recovery/Interpolation Control ==
  Delta : Inport  OutDataTypeStr=fixdt(1, 16, 15)  PortDimensions=1  SampleTime=5e-07
  Interpolation Control : MATLAB Function
  Underflow : Outport  SampleTime=5e-07  VectorParamsAs1DForOutWhenUnconnected=off
  mu : Outport  Port=2  SampleTime=5e-07  VectorParamsAs1DForOutWhenUnconnected=off
  wires:
  Interpolation Control/2(mu) -> mu/1
  Delta/1 -> Interpolation Control/1(Delta)
  Interpolation Control/1(Underflow) -> Underflow/1

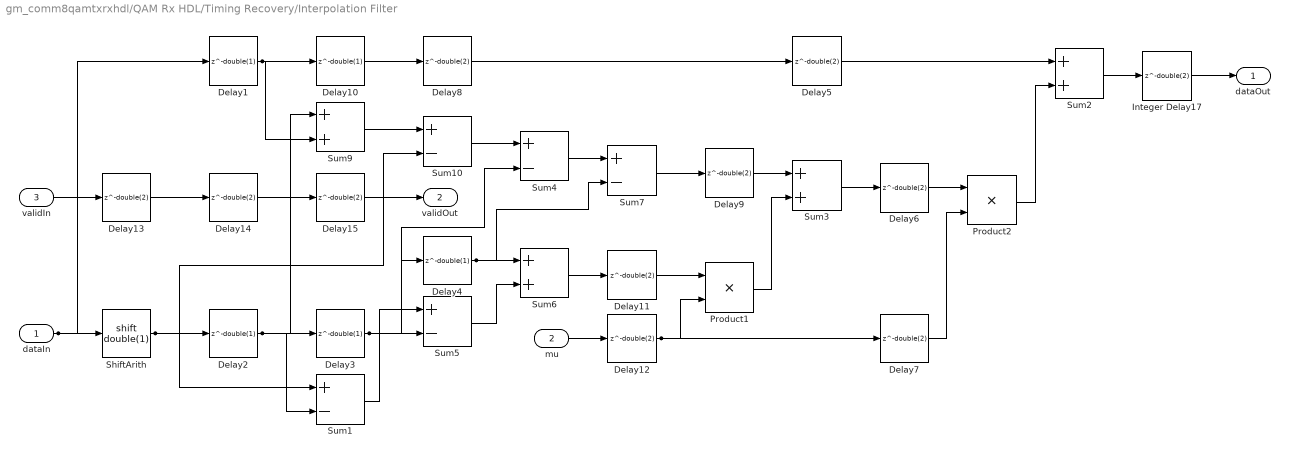
== system gm_comm8qamtxrxhdl/QAM Rx HDL/Timing Recovery/Interpolation Filter  ==
  dataIn : Inport  OutDataTypeStr=fixdt(1, 16, 15)  PortDimensions=1  SampleTime=5e-07
      settings: SignalType=complex
  mu : Inport  Port=2  OutDataTypeStr=fixdt(1, 16, 15)  PortDimensions=1  SampleTime=5e-07
  validIn : Inport  Port=3  OutDataTypeStr=boolean  PortDimensions=1  SampleTime=5e-07
  Delay{1..4,10} (5 alike) : Delay  DelayLength=double(1)  InitialCondition=0  SampleTime=5e-07
  Delay{5..9,11..15} (10 alike) : Delay  DelayLength=double(2)  InitialCondition=0  SampleTime=5e-07
  Integer Delay17 : Delay  DelayLength=double(2)  InitialCondition=0  SampleTime=5e-07
  Product1 : Product  Inputs=**  OutDataTypeStr=fixdt(1, 16, 14)  RndMeth=Zero  SampleTime=5e-07
  Product2 : Product  Inputs=**  OutDataTypeStr=fixdt(1, 16, 14)  RndMeth=Zero  SampleTime=5e-07
  ShiftArith : ArithShift  BitShiftNumber=double(1)  BinPtShiftNumber=double(0)
  Sum1 : Sum  Inputs=+-  OutDataTypeStr=fixdt(1, 16, 14)  AccumDataTypeStr=fixdt(1, 17, 15)  SampleTime=5e-07
  Sum{4..5,7,10} (4 alike) : Sum  Inputs=+-  OutDataTypeStr=fixdt(1, 16, 14)  AccumDataTypeStr=fixdt(1, 18, 15)  SampleTime=5e-07
  Sum2 : Sum  OutDataTypeStr=fixdt(1, 16, 15)  AccumDataTypeStr=fixdt(1, 16, 15)  SampleTime=5e-07
  Sum3 : Sum  OutDataTypeStr=fixdt(1, 17, 14)  AccumDataTypeStr=fixdt(1, 17, 14)  SampleTime=5e-07
  Sum6 : Sum  OutDataTypeStr=fixdt(1, 16, 14)  AccumDataTypeStr=fixdt(1, 18, 15)  SaturateOnIntegerOverflow=on  SampleTime=5e-07
  Sum9 : Sum  OutDataTypeStr=fixdt(1, 16, 14)  AccumDataTypeStr=fixdt(1, 17, 15)  SampleTime=5e-07
  dataOut : Outport  SampleTime=5e-07  VectorParamsAs1DForOutWhenUnconnected=off
  validOut : Outport  Port=2  SampleTime=5e-07  VectorParamsAs1DForOutWhenUnconnected=off
  wires:
  Delay10/1 -> Delay8/1
  validIn/1 -> Delay13/1
  Delay2/1 -> Sum1/2, Sum9/1, Delay3/1
  Delay6/1 -> Product2/1
  Delay1/1 -> Sum9/2, Delay10/1
  dataIn/1 -> Delay1/1, ShiftArith/1
  Delay12/1 -> Delay7/1, Product1/2
  Sum10/1 -> Sum4/1
  Delay13/1 -> Delay14/1
  ShiftArith/1 -> Sum1/1, Sum10/2, Delay2/1
  Sum2/1 -> Integer Delay17/1
  Delay14/1 -> Delay15/1
  Sum9/1 -> Sum10/1
  Delay15/1 -> validOut/1
  Delay3/1 -> Sum4/2, Sum5/2, Delay4/1
  Sum1/1 -> Sum5/1
  Product2/1 -> Sum2/2
  Delay4/1 -> Sum7/2, Sum6/1
  Delay8/1 -> Delay5/1
  Sum5/1 -> Sum6/2
  Integer Delay17/1 -> dataOut/1
  Sum4/1 -> Sum7/1
  Sum6/1 -> Delay11/1
  mu/1 -> Delay12/1
  Sum7/1 -> Delay9/1
  Delay11/1 -> Product1/1
  Delay9/1 -> Sum3/1
  Product1/1 -> Sum3/2
  Delay7/1 -> Product2/2
  Delay5/1 -> Sum2/1
  Sum3/1 -> Delay6/1

== system gm_comm8qamtxrxhdl/QAM Rx HDL/Timing Recovery/Timing Error Detector ==
  In : Inport  OutDataTypeStr=fixdt(1, 16, 15)  PortDimensions=1  SampleTime=5e-07
      settings: SignalType=complex
  strobe : Inport  Port=2  OutDataTypeStr=boolean  PortDimensions=1  SampleTime=5e-07
  Timing Error Detector : MATLAB Function  TreatAsAtomicUnit=on
  e : Outport  SampleTime=5e-07  VectorParamsAs1DForOutWhenUnconnected=off
  wires:
  strobe/1 -> Timing Error Detector/2(strobe)
  In/1 -> Timing Error Detector/1(In)
  Timing Error Detector/1(e) -> e/1

== system gm_comm8qamtxrxhdl/QAM Tx HDL/Data Generation & Packetization/Data Source ==
  reset preamble : Inport
  load preamble : Inport  Port=2
  load data : Inport  Port=3
  Data Address Counter : hdlsllib/Sources/HDL Counter  CountType=Count limited  CountInit=0  CountStep=1  CountMax=qam_params.total_data_bits-1  CountFromType=Initial value  CountFrom=0  CountResetPort=off  CountLoadPort=off  CountEnbPort=on  CountDirPort=off  CountHitOutputPort=off  CountDataType=Unsigned  CountWordLen=16  CountFracLen=0  CountSampTime=1
  HDL Data Scrambler : Subsystem  TreatAsAtomicUnit=on
  Logical Operator : Logic  Operator=NOT  AllPortsSameDT=off  OutDataTypeStr=boolean
  Pipeline : Delay  InitialCondition=0
  Pipeline1 : Delay  InitialCondition=0
  Pipeline2 : Delay  DelayLength=1  InitialCondition=0
  Pipeline3 : Delay  DelayLength=1  InitialCondition=0
  Pipeline4 : Delay  DelayLength=1  InitialCondition=0
  Preamble Address Counter : hdlsllib/Sources/HDL Counter  CountType=Count limited  CountInit=0  CountStep=1  CountMax=128  CountFromType=Initial value  CountFrom=0  CountResetPort=on  CountLoadPort=off  CountEnbPort=on  CountDirPort=off  CountHitOutputPort=off  CountDataType=Unsigned  CountWordLen=16  CountFracLen=0  CountSampTime=1
  Preamble Data Mux : Switch  Criteria=u2 ~= 0  SaturateOnIntegerOverflow=off  InputSameDT=off
  data lookup : LookupNDDirect  NumberOfTableDimensions=1  Table=qam_params.tx_data_bits  DiagnosticForOutOfRangeInput=Error  SampleTime=1/qam_params.bitRate  TableDataTypeStr=boolean
  preamble lookup : LookupNDDirect  NumberOfTableDimensions=1  Table=qam_params.preamble_bits  DiagnosticForOutOfRangeInput=Error  SampleTime=1/qam_params.bitRate  TableDataTypeStr=boolean
  packet_bits : Outport  VectorParamsAs1DForOutWhenUnconnected=off
  wires:
  reset preamble/1 -> Preamble Address Counter/1
  Preamble Address Counter/1 -> preamble lookup/1
  HDL Data Scrambler/1(Scrambled_Out) -> Pipeline4/1
  Pipeline2/1 -> HDL Data Scrambler/Enable
  Data Address Counter/1 -> data lookup/1
  data lookup/1 -> Pipeline3/1
  Pipeline3/1 -> HDL Data Scrambler/1(Data_In)
  preamble lookup/1 -> Pipeline/1
  Pipeline4/1 -> Preamble Data Mux/3
  Pipeline/1 -> Preamble Data Mux/1
  Pipeline1/1 -> Preamble Data Mux/2
  Preamble Data Mux/1 -> packet_bits/1
  load data/1 -> Data Address Counter/1, Logical Operator/1, Pipeline2/1
  load preamble/1 -> Preamble Address Counter/2
  Logical Operator/1 -> Pipeline1/1

== system gm_comm8qamtxrxhdl/QAM Tx HDL/Data Generation & Packetization/Group Bits ==
  Bits In : Inport
  Bit Concat : hdlsllib/Logic and Bit Operations/Bit Concat  numInputs=3
  Delay4 : Delay  InitialCondition=0
  Delay5 : Delay  DelayLength=1  InitialCondition=0
  Downsample : DownSample  N=3  phase=2  RateOptions=Allow multirate processing
  Integer Out : Outport  VectorParamsAs1DForOutWhenUnconnected=off
  wires:
  Downsample/1 -> Integer Out/1
  Bit Concat/1 -> Downsample/1
  Delay5/1 -> Bit Concat/2
  Delay4/1 -> Bit Concat/1
  Bits In/1 -> Bit Concat/3, Delay5/1, Delay4/1

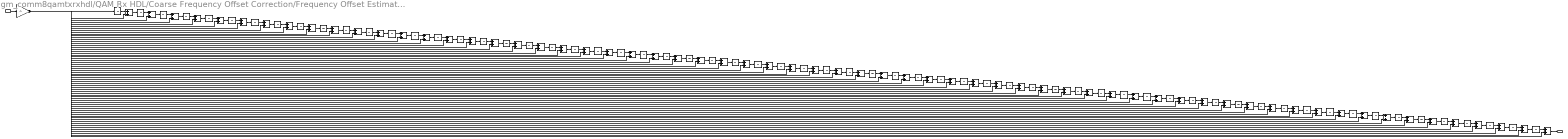
== system gm_comm8qamtxrxhdl/QAM Rx HDL/Coarse Frequency Offset Correction/Frequency Offset Estimation/Discrete FIR Filter ==
  Discrete FIR Filter_in : Inport  OutDataTypeStr=fixdt(1, 16, 15)  SampleTime=5e-07
      settings: SignalType=complex
  adder{0..62} (63 alike) : Sum  OutDataTypeStr=fixdt(1, 19, 15)  SampleTime=5e-07
  gain63 : Gain  Gain="fi(0,1,2,0,\"hex\",\"1\")"  ParamDataTypeStr=fixdt(1, 2, 0)  OutDataTypeStr=fixdt(1, 16, 15)  SampleTime=5e-07
  unit_delay{,1..62} (63 alike) : UnitDelay  InitialCondition=double(0)  SampleTime=5e-07
  Discrete FIR Filter_out : Outport  OutDataTypeStr=fixdt(1, 19, 15)  SampleTime=5e-07
      settings: SignalType=complex
  wires:
  adder32/1 -> unit_delay32/1
  adder44/1 -> unit_delay44/1
  unit_delay17/1 -> adder16/1
  adder12/1 -> unit_delay12/1
  adder20/1 -> unit_delay20/1
  adder52/1 -> unit_delay52/1
  adder36/1 -> unit_delay36/1
  unit_delay49/1 -> adder48/1
  adder23/1 -> unit_delay23/1
  adder55/1 -> unit_delay55/1
  adder11/1 -> unit_delay11/1
  adder43/1 -> unit_delay43/1
  unit_delay58/1 -> adder57/1
  unit_delay41/1 -> adder40/1
  adder30/1 -> unit_delay30/1
  adder62/1 -> unit_delay62/1
  adder29/1 -> unit_delay29/1
  adder61/1 -> unit_delay61/1
  adder28/1 -> unit_delay28/1
  adder60/1 -> unit_delay60/1
  unit_delay37/1 -> adder36/1
  adder27/1 -> unit_delay27/1
  adder59/1 -> unit_delay59/1
  unit_delay45/1 -> adder44/1
  adder33/1 -> unit_delay33/1
  unit_delay33/1 -> adder32/1
  adder24/1 -> unit_delay24/1
  adder56/1 -> unit_delay56/1
  unit_delay21/1 -> adder20/1
  adder15/1 -> unit_delay15/1
  adder47/1 -> unit_delay47/1
  adder26/1 -> unit_delay26/1
  adder58/1 -> unit_delay58/1
  adder25/1 -> unit_delay25/1
  adder57/1 -> unit_delay57/1
  adder22/1 -> unit_delay22/1
  adder54/1 -> unit_delay54/1
  adder1/1 -> unit_delay1/1
  adder5/1 -> unit_delay5/1
  unit_delay29/1 -> adder28/1
  adder21/1 -> unit_delay21/1
  adder53/1 -> unit_delay53/1
  adder19/1 -> unit_delay19/1
  adder51/1 -> unit_delay51/1
  unit_delay7/1 -> adder6/1
  adder34/1 -> unit_delay34/1
  unit_delay25/1 -> adder24/1
  adder18/1 -> unit_delay18/1
  adder50/1 -> unit_delay50/1
  adder17/1 -> unit_delay17/1
  adder49/1 -> unit_delay49/1
  unit_delay57/1 -> adder56/1
  adder42/1 -> unit_delay42/1
  adder10/1 -> unit_delay10/1
  adder16/1 -> unit_delay16/1
  adder48/1 -> unit_delay48/1
  adder14/1 -> unit_delay14/1
  adder46/1 -> unit_delay46/1
  unit_delay62/1 -> adder61/1
  adder13/1 -> unit_delay13/1
  adder45/1 -> unit_delay45/1
  unit_delay61/1 -> adder60/1
  adder40/1 -> unit_delay40/1
  unit_delay13/1 -> adder12/1
  adder9/1 -> unit_delay9/1
  adder41/1 -> unit_delay41/1
  unit_delay53/1 -> adder52/1
  adder39/1 -> unit_delay39/1
  unit_delay52/1 -> adder51/1
  adder38/1 -> unit_delay38/1
  unit_delay48/1 -> adder47/1
  adder37/1 -> unit_delay37/1
  adder35/1 -> unit_delay35/1
  adder2/1 -> unit_delay2/1
  adder31/1 -> unit_delay31/1
  adder8/1 -> unit_delay8/1
  adder7/1 -> unit_delay7/1
  adder6/1 -> unit_delay6/1
  adder4/1 -> unit_delay4/1
  adder3/1 -> unit_delay3/1
  unit_delay60/1 -> adder59/1
  unit_delay59/1 -> adder58/1
  unit_delay56/1 -> adder55/1
  unit_delay55/1 -> adder54/1
  unit_delay54/1 -> adder53/1
  unit_delay51/1 -> adder50/1
  unit_delay50/1 -> adder49/1
  unit_delay47/1 -> adder46/1
  unit_delay46/1 -> adder45/1
  unit_delay9/1 -> adder8/1
  unit_delay44/1 -> adder43/1
  unit_delay43/1 -> adder42/1
  unit_delay42/1 -> adder41/1
  unit_delay40/1 -> adder39/1
  unit_delay39/1 -> adder38/1
  unit_delay38/1 -> adder37/1
  unit_delay36/1 -> adder35/1
  unit_delay35/1 -> adder34/1
  unit_delay28/1 -> adder27/1
  unit_delay34/1 -> adder33/1
  unit_delay32/1 -> adder31/1
  gain63/1 -> adder1/2, adder2/2, adder7/2, adder15/2, adder12/2, adder16/2, adder13/2, adder6/2, adder19/2, adder20/2, adder21/2, adder23/2, adder26/2, adder27/2, adder28/2, adder10/2, adder30/2, adder32/2, adder34/2, adder31/2, adder9/2, adder39/2, adder40/2, adder5/2, adder0/2, adder42/2, adder29/2, adder43/2, adder8/2, adder44/2, adder45/2, adder25/2, adder22/2, adder46/2, adder47/2, adder48/2, adder37/2, adder24/2, adder17/2, adder49/2, adder50/2, adder3/2, adder51/2, adder38/2, adder33/2, adder53/2, adder57/2, adder36/2, adder59/2, adder55/2, adder41/2, adder14/2, adder56/2, adder60/2, adder35/2, adder58/2, adder4/2, adder61/2, adder11/2, adder62/2, adder18/2, adder52/2, unit_delay/1, adder54/2
  unit_delay31/1 -> adder30/1
  unit_delay30/1 -> adder29/1
  unit_delay27/1 -> adder26/1
  unit_delay26/1 -> adder25/1
  unit_delay24/1 -> adder23/1
  unit_delay23/1 -> adder22/1
  unit_delay22/1 -> adder21/1
  unit_delay20/1 -> adder19/1
  unit_delay19/1 -> adder18/1
  unit_delay6/1 -> adder5/1
  unit_delay18/1 -> adder17/1
  unit_delay16/1 -> adder15/1
  unit_delay15/1 -> adder14/1
  unit_delay14/1 -> adder13/1
  unit_delay12/1 -> adder11/1
  unit_delay11/1 -> adder10/1
  unit_delay10/1 -> adder9/1
  unit_delay8/1 -> adder7/1
  unit_delay5/1 -> adder4/1
  unit_delay4/1 -> adder3/1
  unit_delay3/1 -> adder2/1
  unit_delay2/1 -> adder1/1
  unit_delay1/1 -> adder0/1
  unit_delay/1 -> adder62/1
  adder0/1 -> Discrete FIR Filter_out/1
  Discrete FIR Filter_in/1 -> gain63/1

== system gm_comm8qamtxrxhdl/QAM Rx HDL/Coarse Frequency Offset Correction/Frequency Offset Estimation/Enabled Wire ==
  In1 : Inport  OutDataTypeStr=fixdt(1, 32, 31)  PortDimensions=1  SampleTime=5e-07
      settings: SignalType=complex
  Enable : Inport  Port=2  OutDataTypeStr=boolean  SampleTime=5e-07
  In1bypassMux : Switch  Criteria=u2 ~= 0  Threshold=double(0)  OutDataTypeStr=fixdt(1, 32, 31)  SampleTime=5e-07  SaturateOnIntegerOverflow=off  InputSameDT=off
  Out1_bypass : UnitDelay  InitialCondition="fi(0,1,32,31,\"hex\",\"00000000\")"  SampleTime=5e-07
  Out1 : Outport  SampleTime=5e-07  InitialOutput=0  VectorParamsAs1DForOutWhenUnconnected=off
  wires:
  Out1_bypass/1 -> In1bypassMux/3
  In1/1 -> In1bypassMux/1
  Enable/1 -> In1bypassMux/2
  In1bypassMux/1 -> Out1_bypass/1, Out1/1
